simulink model "sf_frame_sync_controller"  (R2025b)
settings: Solver=FixedStepDiscrete  StartTime=0.0  StopTime=15  FixedStep=0.05  RelTol=1e-3  EnableMultiTasking=on
model workspace (MAT data in the model file):
  trainSig = [-0.707106781187+0.707106781187i; -0.707106781187+0.707106781187i; -0.707106781187+0.707106781187i; -0.707106781187+0.707106781187i; -0.707106781187-0.707106781187i; -0.707106781187-0.707106781187i; 0.707106781187-0.707106781187i; 0.707106781187-0.707106781187i; -0.707106781187-0.707106781187i; -0.707106781187+0.707106781187i; 0.707106781187-0.707106781187i; -0.707106781187-0.707106781187i; -0.707106781187+0.707106781187i; 0.707106781187-0.707106781187i; 0.707106781187-0.707106781187i; -0.707106781187-0.707106781187i; -0.707106781187-0.707106781187i; -0.707106781187-0.707106781187i; 0.707106781187+0.707106781187i; -0.707106781187+0.707106781187i; -0.707106781187+0.707106781187i; 0.707106781187+0.707106781187i; 0.707106781187-0.707106781187i; 0.707106781187+0.707106781187i; 0.707106781187+0.707106781187i; 0.707106781187+0.707106781187i; 0.707106781187+0.707106781187i; -0.707106781187+0.707106781187i; -0.707106781187+0.707106781187i; 0.707106781187-0.707106781187i; -0.707106781187+0.707106781187i; 0.707106781187+0.707106781187i; 0.707106781187-0.707106781187i; 0.707106781187-0.707106781187i; -0.707106781187+0.707106781187i; 0.707106781187+0.707106781187i; -0.707106781187+0.707106781187i; -0.707106781187+0.707106781187i; -0.707106781187-0.707106781187i; -0.707106781187+0.707106781187i; -0.707106781187-0.707106781187i; -0.707106781187-0.707106781187i; 0.707106781187+0.707106781187i; 0.707106781187+0.707106781187i; -0.707106781187+0.707106781187i; -0.707106781187+0.707106781187i; -0.707106781187+0.707106781187i; -0.707106781187-0.707106781187i; 0.707106781187+0.707106781187i; -0.707106781187+0.707106781187i; 0.707106781187-0.707106781187i; 0.707106781187+0.707106781187i; 0.707106781187-0.707106781187i; -0.707106781187-0.707106781187i; -0.707106781187+0.707106781187i; -0.707106781187-0.707106781187i; 0.707106781187+0.707106781187i; -0.707106781187+0.707106781187i; 0.707106781187-0.707106781187i; -0.707106781187-0.707106781187i; -0.707106781187-0.707106781187i; 0.707106781187+0.707106781187i; -0.707106781187+0.707106781187i; -0.707106781187-0.707106781187i]
settings Model: Creator=The MathWorks, Inc.  LastModifiedBy=The MathWorks, Inc.
settings SolverCC: AlgebraicLoopSolver=TrustRegion
settings DataIOCC: LimitDataPoints=on  SaveFormat=StructureWithTime  SaveOutput=off  SignalLogging=off  SaveTime=off  ReturnWorkspaceOutputs=off
settings OptimizationCC: ReuseModelBlockBuffer=off  ExpressionDepthLimit=2147483647.0  InitFltsAndDblsToZero=on  EfficientMapNaN2IntZero=off  LifeSpan=inf
settings DebuggingCC: UnderspecifiedInitializationDetection=Classic  MergeDetectMultiDrivingBlocksExec=none  FcnCallInpInsideContextMsg=warning  UnconnectedInputMsg=warning  UnconnectedOutputMsg=warning  UnconnectedLineMsg=warning  StateNameClashWarn=warning  SFUnexpectedBacktrackingDiag=warning  SFNoUnconditionalDefaultTransitionDiag=warning  SFExecutionAtInitializationDiag=none  ArithmeticOperatorsInVariantConditions=warning
settings HardwareCC: ProdBitPerPointer=32.0  ProdBitPerSizeT=32.0  ProdBitPerPtrDiffT=32.0  ProdLargestAtomicFloat=None  ProdIntDivRoundTo=Undefined  ProdEndianess=Unspecified  ProdWordSize=32.0  ProdHWDeviceType=32-bit Generic
settings ModelReferenceCC: EnableRefExpFcnMdlSchedulingChecks=on  PropagateSignalLabelsOutOfModel=off
settings SFSimCC: SimUseLocalCustomCode=off  SimParseCustomCode=off  CustomCodeUndefinedFunction=UseInterfaceOnly
settings RTWCC: RTWUseLocalCustomCode=off  GPUComputeCapability=3.5
settings CodeAppCC: StateflowObjectComments=on
settings GRTTargetCC: TargetLangStandard=C89/C90 (ANSI)  CombineOutputUpdateFcns=off  GRTInterface=on
settings ConfigComp: CovMetricSettings=dw  CovSaveCumulativeToWorkspaceVar=on  CovSaveSingleToWorkspaceVar=on  CovExternalEMLEnable=off  CovSFcnEnable=off

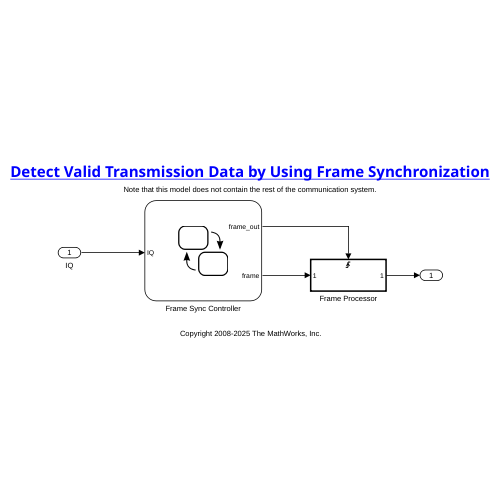
[thumbnail: Simulink's stored preview of the top-level diagram]
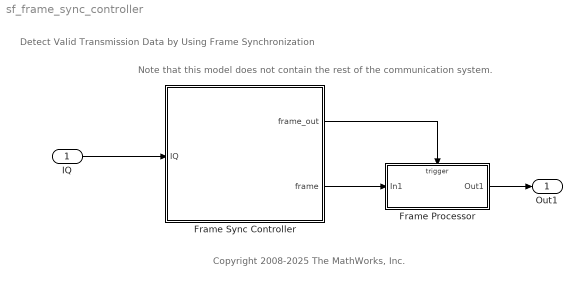
== system sf_frame_sync_controller ==
  note: Note that this model does not contain the rest of the communication system.
  note: Copyright 2008-2025 The MathWorks, Inc.
  note: Detect Valid Transmission Data by Using Frame Synchronization
  IQ : Inport
  Frame Processor : Subsystem  TreatAsAtomicUnit=on
  Frame Sync Controller : Stateflow chart  TreatAsAtomicUnit=on
  Out1 : Outport  VectorParamsAs1DForOutWhenUnconnected=off
  wires:
  IQ/1 -> Frame Sync Controller/1(IQ)
  Frame Sync Controller/2(frame) -> Frame Processor/1(In1)
  Frame Sync Controller/1(" frame_out") -> Frame Processor/Trigger
  Frame Processor/1(Out1) -> Out1/1

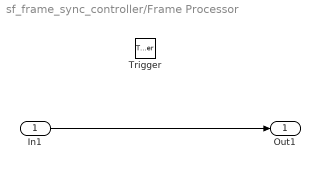
== system sf_frame_sync_controller/Frame Processor ==
  In1 : Inport
  Trigger : TriggerPort  VariantControl=(inherit)
  Out1 : Outport  VectorParamsAs1DForOutWhenUnconnected=off
  wires:
  In1/1 -> Out1/1

== stateflow chart sf_frame_sync_controller/Frame Sync Controller ==
  state look_for_sync
    en:
    corrAbs = 0;
    du:
    [corr, corrAbs] = correlate(IQ);
  state frame_out
  state get_payload
    en:
    phasor = get_carrier_phase(corr);
    frame[0] = IQ*phasor;
    du:
    frame[count(true)] = IQ*phasor;
  (default) -> look_for_sync
  frame_out -> look_for_sync
  look_for_sync -> frame_out [order 2] : [after(300,tick)]
      | {frame = 0;}
  look_for_sync -> get_payload [order 1] : [corrAbs > 50]
  get_payload -> frame_out : [after(220,tick)]
  data: u function_input double; y function_output double; yabs function_output double; u function_input double; y function_output double; IQ input double; phasor local double; corr local double; corrAbs local double; frame_out output boolean; frame output double size=221; trainSig local double size=64
  function [y, yabs] = correlate(u):
    | function [y, yabs] = correlate(u)
    | 
    | persistent zi;
    | 
    | B = conj(flipud(trainSig));
    | A = 1;
    | 
    | if(isempty(zi))
    |     zi = zeros(max(length(A),length(B))-1,1) + complex(0,0);
    | end
    | 
    | [y,zi] = filter(B,A,u,zi);
    | 
    | yabs = abs(y);
  function y = get_carrier_phase(u):
    | function y = get_carrier_phase(u)
    | 
    | y = exp(-1i*angle(u));
